simulink model "sm_cvt_power_split_pg_4range"  (R2025a)
settings: Solver=daessc  StartTime=0.0  StopTime=cvtPar.ratioInp.t(end)  MaxStep=0.01  RelTol=1e-3  AbsTol=1e-4  EnableMultiTasking=on
PreLoadFcn:
  | cvtPar = sm_cvt_power_split_pg_4range_param('InputOutput', HMPST);
PostLoadFcn:
  | set_param([bdroot '/Manual Switch'], 'sw', '1')
StartFcn:
  | tic
StopFcn:
  | Elapsed_Sim_Time = toc;
  | disp(['Elapsed Sim Time = ' num2str(Elapsed_Sim_Time)]);
values from neighbouring files (symbols this model uses):
  HMPST = varargin{2}    [sm_cvt_power_split_pg_4range_param.m]
undefined symbols (not defined in the file or in its folder): Local, X, Y, Z
libraries: sm_lib x37, fl_lib x22, nesl_utility x10, planetary_gear_lib x9, Multibody_Parts_Lib x8, simulink x2, sm_wheel_loader_lib x1
(part 1 of 2)
CloseFcn:
  | try,close(h1_sm_planetary_gear_testrig),end
  | clear h1_sm_planetary_gear_testrig
  | 
  | clear simlog_sm_planetary_gear_testrig
  | clear logsout_sm_planetary_gear_testrig
Description:
  | Power Split CVT with Four Speed Ranges
  | 
  | Copyright 2023-2025 The MathWorks, Inc.
settings Model: Creator=smiller  LastModifiedBy=smiller
settings SolverCC: AutoScaleAbsTol=off  AlgebraicLoopSolver=TrustRegion
settings DataIOCC: MaxDataPoints=20000  SaveFormat=Array  ReturnWorkspaceOutputs=off  SignalLoggingName=logsout_sm_cvt_power_split_pg_4range
settings OptimizationCC: ReuseModelBlockBuffer=off  LifeSpan=inf
settings DebuggingCC: UnderspecifiedInitializationDetection=Classic  MergeDetectMultiDrivingBlocksExec=none  SolverPrmCheckMsg=warning  UnconnectedInputMsg=warning  UnconnectedOutputMsg=warning  UnconnectedLineMsg=warning  StateNameClashWarn=warning  PregeneratedLibrarySubsystemCodeDiagnostic=none  SFUnexpectedBacktrackingDiag=warning  SFNoUnconditionalDefaultTransitionDiag=warning  SFExecutionAtInitializationDiag=none  ArithmeticOperatorsInVariantConditions=warning
settings HardwareCC: ProdBitPerPointer=32.0  ProdBitPerSizeT=32.0  ProdBitPerPtrDiffT=32.0  ProdLargestAtomicFloat=None  ProdIntDivRoundTo=Undefined  ProdEndianess=Unspecified  ProdWordSize=32.0  ProdHWDeviceType=32-bit Generic
settings ModelReferenceCC: EnableRefExpFcnMdlSchedulingChecks=on  PropagateSignalLabelsOutOfModel=off
settings SFSimCC: SimUseLocalCustomCode=off  CustomCodeUndefinedFunction=UseInterfaceOnly
settings RTWCC: RTWUseLocalCustomCode=off  GPUComputeCapability=3.5  DLArmComputeVersion=19.05
settings CodeAppCC: StateflowObjectComments=on
settings GRTTargetCC: TargetLangStandard=C89/C90 (ANSI)
settings ConfigComp: CovMetricSettings=dw  CovSaveCumulativeToWorkspaceVar=on  CovSaveSingleToWorkspaceVar=on  CovExternalEMLEnable=off
settings SimscapeCC: SimscapeNormalizeSystem=off  SimscapeLogType=all  SimscapeLogSimulationStatistics=on  SimscapeLogName=simlog_sm_cvt_power_split_pg_4range  SimscapeLogLimitData=off  SimscapeLogDataHistory=20000.0
settings ConfigurationSet: Description=SimMechanics 2G
settings DiagnosticsConfigSet: SimMechanicsUnconnectedFramePorts=none
settings ExplorerConfigSet: InternalSimMechanicsExplorerSettings="<ExplorerConfiguration><canonicalview>default</canonicalview><AnimationSetting><BasePlaybackSpeed>1.0</BasePlaybackSpeed><PlaybackSpeedFactor>2.0</PlaybackSpeedFactor></AnimationSetting><TilePanel><TileInfo><Tiles Columns=\"1\" Count=\"1\" Rows=\"1\"><Column Weight=\"1\"/><Row Weight=\"1\"/><Tile Height=\"1\" Width=\"1\" X=\"0\" Y=\"0\"/></Tiles></TileInfo><SceneInfo><SceneViewer><BGColor><R>1</R><G>1</G><B>1</B></BGColor><Camera><DoPerspective>off</DoPerspective><Position><X>0.0480133750302565443</X><Y>0.998189165564586478</Y><Z>0.410806874332134753</Z></Position><Center><X>0.0475311378746693936</X><Y>0.0361071202127969879</Y><Z>0.138047079899298764</Z></Center><Up><X>0.999999473002182615</X><Y>-0.000216739834242075458</Y><Z>-0.0010035034634835007</Z></Up><ViewLimDist>1</ViewLimDist><YLim>0.276201890267888606</YLim><XLim>0.56263348017532866</XLim></Camera></SceneViewer></SceneInfo></TilePanel><MechEditorPanel><Cameras/><GfxPanelCameraMap/><VideoCreator><PlaybackSpeedRatio>2</PlaybackSpeedRatio><FrameRate>30</FrameRate><VideoFormat>MPEG-4</VideoFormat><FrameSize>auto</FrameSize></VideoCreator></MechEditorPanel></ExplorerConfiguration>"

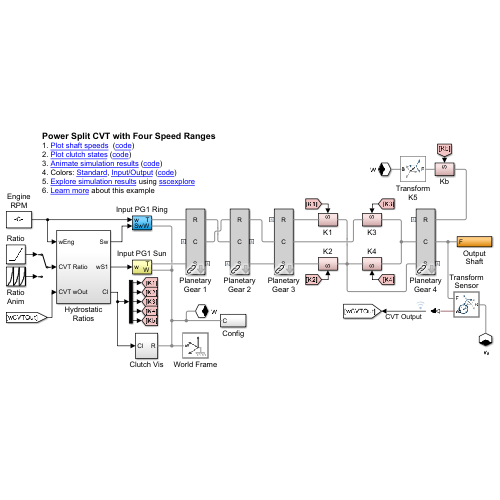
[thumbnail: Simulink's stored preview of the top-level diagram]
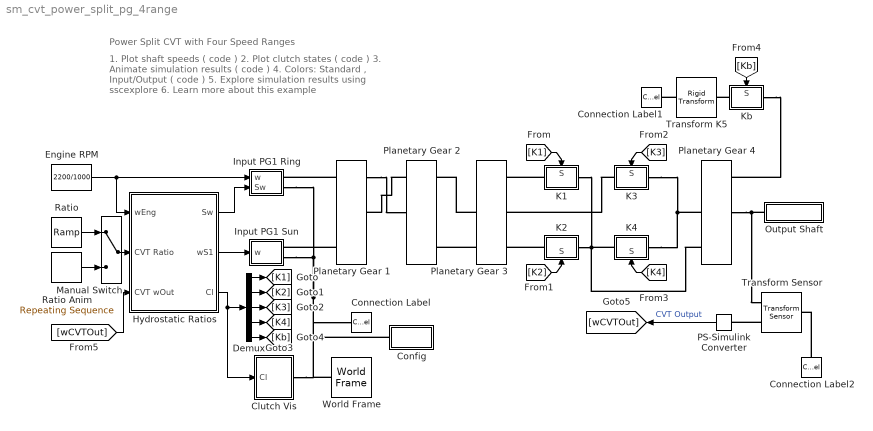
== system sm_cvt_power_split_pg_4range ==
  note: Power Split CVT with Four Speed Ranges
  note: 1. Plot shaft speeds ( code )
      | 2. Plot clutch states ( code )
      | 3. Animate simulation results ( code )
      | 4. Colors: Standard , Input/Output ( code )
      | 5. Explore simulation results using sscexplore
      | 6. Learn more about this example
  Clutch Vis : Subsystem
  Config : Subsystem
  Connection Label : ConnectionLabel  Label=W
  Connection Label1 : ConnectionLabel  Label=W
  Connection Label2 : ConnectionLabel  Label=W
  Demux : Demux  Outputs=5
  Engine RPM : Constant  Value=2200/1000
  Hydrostatic Ratios : Subsystem
  Input PG1 Ring : Subsystem  Tag=PublishSubsystem
  Input PG1 Sun : Subsystem  Tag=PublishSubsystem
  K1 : Subsystem
      settings: PortSchema="{\"entries\":[{\"content\":{\"sides\":[{\"content\":{\"connectorIds\":[\"LConn1\"]},\"type\":\"ConnectorPlacement.EquallySpacedRectSide\",\"uuid\":\"8540058f-cef1-4155-b235-6fcdc2adbf7a\"},{\"content\":{\"connectorIds\":[\"RConn1\"],\"side\":\"RIGHT\"},\"type\":\"ConnectorPlacement.EquallySpacedRectSide\",\"uuid\":\"a5955f9a-e2a5-407c-ab0f-07844d9b5a94\"},{\"content\":{\"connectorIds\":[\"In1\"],\"side\":\"TOP\"},\"type\":\"ConnectorPlacement.EquallySpacedRectSide\",\"uuid\":\"6ad60a3a-82ac-4ebb-acab-e8d6af80f4b1\"}]},\"type\":\"ConnectorPlacement.EquallySpacedConnector\",\"uuid\":\"9d3f1ab8-7892-4728-ac99-ab2f347c5259\"}],\"packageUris\":[\"http://schema.mathworks.com/mf0/Connector/R2020b\"],\"version\":\"1.0\"}"
  K2 : Subsystem
      settings: PortSchema="{\"entries\":[{\"content\":{\"sides\":[{\"content\":{\"connectorIds\":[\"LConn1\"]},\"type\":\"ConnectorPlacement.EquallySpacedRectSide\",\"uuid\":\"8540058f-cef1-4155-b235-6fcdc2adbf7a\"},{\"content\":{\"connectorIds\":[\"RConn1\"],\"side\":\"RIGHT\"},\"type\":\"ConnectorPlacement.EquallySpacedRectSide\",\"uuid\":\"a5955f9a-e2a5-407c-ab0f-07844d9b5a94\"},{\"content\":{\"connectorIds\":[\"In1\"],\"side\":\"TOP\"},\"type\":\"ConnectorPlacement.EquallySpacedRectSide\",\"uuid\":\"6ad60a3a-82ac-4ebb-acab-e8d6af80f4b1\"}]},\"type\":\"ConnectorPlacement.EquallySpacedConnector\",\"uuid\":\"9d3f1ab8-7892-4728-ac99-ab2f347c5259\"}],\"packageUris\":[\"http://schema.mathworks.com/mf0/Connector/R2020b\"],\"version\":\"1.0\"}"
  K3 : Subsystem
      settings: PortSchema="{\"entries\":[{\"content\":{\"sides\":[{\"content\":{\"connectorIds\":[\"LConn1\"]},\"type\":\"ConnectorPlacement.EquallySpacedRectSide\",\"uuid\":\"8540058f-cef1-4155-b235-6fcdc2adbf7a\"},{\"content\":{\"connectorIds\":[\"RConn1\"],\"side\":\"RIGHT\"},\"type\":\"ConnectorPlacement.EquallySpacedRectSide\",\"uuid\":\"a5955f9a-e2a5-407c-ab0f-07844d9b5a94\"},{\"content\":{\"connectorIds\":[\"In1\"],\"side\":\"TOP\"},\"type\":\"ConnectorPlacement.EquallySpacedRectSide\",\"uuid\":\"6ad60a3a-82ac-4ebb-acab-e8d6af80f4b1\"}]},\"type\":\"ConnectorPlacement.EquallySpacedConnector\",\"uuid\":\"9d3f1ab8-7892-4728-ac99-ab2f347c5259\"}],\"packageUris\":[\"http://schema.mathworks.com/mf0/Connector/R2020b\"],\"version\":\"1.0\"}"
  K4 : Subsystem
      settings: PortSchema="{\"entries\":[{\"content\":{\"sides\":[{\"content\":{\"connectorIds\":[\"LConn1\"]},\"type\":\"ConnectorPlacement.EquallySpacedRectSide\",\"uuid\":\"8540058f-cef1-4155-b235-6fcdc2adbf7a\"},{\"content\":{\"connectorIds\":[\"RConn1\"],\"side\":\"RIGHT\"},\"type\":\"ConnectorPlacement.EquallySpacedRectSide\",\"uuid\":\"a5955f9a-e2a5-407c-ab0f-07844d9b5a94\"},{\"content\":{\"connectorIds\":[\"In1\"],\"side\":\"TOP\"},\"type\":\"ConnectorPlacement.EquallySpacedRectSide\",\"uuid\":\"6ad60a3a-82ac-4ebb-acab-e8d6af80f4b1\"}]},\"type\":\"ConnectorPlacement.EquallySpacedConnector\",\"uuid\":\"9d3f1ab8-7892-4728-ac99-ab2f347c5259\"}],\"packageUris\":[\"http://schema.mathworks.com/mf0/Connector/R2020b\"],\"version\":\"1.0\"}"
  Kb : Subsystem
      settings: PortSchema="{\"entries\":[{\"content\":{\"sides\":[{\"content\":{\"connectorIds\":[\"LConn1\"]},\"type\":\"ConnectorPlacement.EquallySpacedRectSide\",\"uuid\":\"8540058f-cef1-4155-b235-6fcdc2adbf7a\"},{\"content\":{\"connectorIds\":[\"RConn1\"],\"side\":\"RIGHT\"},\"type\":\"ConnectorPlacement.EquallySpacedRectSide\",\"uuid\":\"a5955f9a-e2a5-407c-ab0f-07844d9b5a94\"},{\"content\":{\"connectorIds\":[\"In1\"],\"side\":\"TOP\"},\"type\":\"ConnectorPlacement.EquallySpacedRectSide\",\"uuid\":\"6ad60a3a-82ac-4ebb-acab-e8d6af80f4b1\"}]},\"type\":\"ConnectorPlacement.EquallySpacedConnector\",\"uuid\":\"9d3f1ab8-7892-4728-ac99-ab2f347c5259\"}],\"packageUris\":[\"http://schema.mathworks.com/mf0/Connector/R2020b\"],\"version\":\"1.0\"}"
  Manual Switch : ManualSwitch
  Output Shaft : Subsystem
  PS-Simulink Converter : nesl_utility/PS-Simulink Converter  PhysicalDomain=network_engine_domain  SubClassName=ps_output  LeftPortType=input  RightPortType=output  PseudoPeriodic=off  Frequencies=[]  VectorFormat=inherit  Unit=rpm  AffineConversion=off
  Planetary Gear 1 : planetary_gear_lib/Planetary Gear  Tag=PublishSubsystem  rad_sun=cvtPar.pg1_sun_rad  nteeth_sun=cvtPar.pg1_sun_nteeth  rad_planet=cvtPar.pg1_pla_rad  nteeth_planet=cvtPar.pg1_pla_nteeth  rad_ring=2*cvtPar.pg1_pla_rad+cvtPar.pg1_sun_rad  nteeth_ring=cvtPar.pg1_rin_nteeth  pg_axial_offset=cvtPar.plaGear_axial_offset*1.25  gear_thickness=cvtPar.gear_thickness  link_thickness=cvtPar.link_thickness  rad_hole=cvtPar.rad_hole  ring_gear_clr=cvtPar.clr.pg1.ring  sun_gear_clr=cvtPar.clr.pg1.sun  pla_gear_clr=cvtPar.clr.pg1.pla  carrier_color=cvtPar.clr.pg1.carr
  Planetary Gear 2 : planetary_gear_lib/Planetary Gear  Tag=PublishSubsystem  rad_sun=cvtPar.pg2_sun_rad  nteeth_sun=cvtPar.pg2_sun_nteeth  rad_planet=cvtPar.pg2_pla_rad  nteeth_planet=cvtPar.pg2_pla_nteeth  rad_ring=2*cvtPar.pg2_pla_rad+cvtPar.pg2_sun_rad  nteeth_ring=cvtPar.pg2_rin_nteeth  pg_axial_offset=cvtPar.plaGear_axial_offset*1.25  gear_thickness=cvtPar.gear_thickness  link_thickness=cvtPar.link_thickness  rad_hole=cvtPar.rad_hole  ring_gear_clr=cvtPar.clr.pg2.ring  sun_gear_clr=cvtPar.clr.pg2.sun  pla_gear_clr=cvtPar.clr.pg2.pla  carrier_color=cvtPar.clr.pg2.carr
  Planetary Gear 3 : planetary_gear_lib/Planetary Gear  Tag=PublishSubsystem  rad_sun=cvtPar.pg3_sun_rad  nteeth_sun=cvtPar.pg3_sun_nteeth  rad_planet=cvtPar.pg3_pla_rad  nteeth_planet=cvtPar.pg3_pla_nteeth  rad_ring=2*cvtPar.pg3_pla_rad+cvtPar.pg3_sun_rad  nteeth_ring=cvtPar.pg3_rin_nteeth  pg_axial_offset=cvtPar.plaGear_axial_offset*3  gear_thickness=cvtPar.gear_thickness  link_thickness=cvtPar.link_thickness  rad_hole=cvtPar.rad_hole  ring_gear_clr=cvtPar.clr.pg3.ring  sun_gear_clr=cvtPar.clr.pg3.sun  pla_gear_clr=cvtPar.clr.pg3.pla  carrier_color=cvtPar.clr.pg3.carr
  Planetary Gear 4 : planetary_gear_lib/Planetary Gear  Tag=PublishSubsystem  rad_sun=cvtPar.pg4_sun_rad  nteeth_sun=cvtPar.pg4_sun_nteeth  rad_planet=cvtPar.pg4_pla_rad  nteeth_planet=cvtPar.pg4_pla_nteeth  rad_ring=2*cvtPar.pg4_pla_rad+cvtPar.pg4_sun_rad  nteeth_ring=cvtPar.pg4_rin_nteeth  pg_axial_offset=cvtPar.plaGear_axial_offset  gear_thickness=cvtPar.gear_thickness  link_thickness=cvtPar.link_thickness  rad_hole=cvtPar.rad_hole  ring_gear_clr=cvtPar.clr.pg4.ring  sun_gear_clr=cvtPar.clr.pg4.sun  pla_gear_clr=cvtPar.clr.pg4.pla  carrier_color=cvtPar.clr.pg4.carr
  Ratio : simulink/Sources/Ramp  slope=cvtPar.ratioInp.r(end)/(cvtPar.ratioInp.t(end)-20)  start=10  InitialOutput=0
  Ratio Anim : simulink/Sources/Repeating Sequence  rep_seq_t=cvtPar.ratioInp.t  rep_seq_y=cvtPar.ratioInp.r
  Transform K5 : sm_lib/Frames and Transforms/Rigid Transform  RotationMethod=None  FollAlignAxisA=+X  BaseAlignAxisA=+Y  FollAlignAxisB=+Y  BaseAlignAxisB=+Z  RotationStandardAxis=+Z  RotationAngle=0.0  RotationAngleUnits=deg  RotationArbitraryAxis=[0 0 1]  RotationSequenceAxes=FollowerAxes  RotationSequence=XYX  RotationSequenceAngles=[0 0 0]  RotationSequenceAnglesUnits=deg  RotationMatrix=[1 0 0; 0 1 0; 0 0 1]  Quaternion=[1 0 0 0]  TranslationMethod=StandardAxis  TranslationCartesianOffset=[0 0 0]  TranslationCartesianOffsetUnits=m  TranslationStandardAxis=+Z  TranslationStandardOffset=cvtPar.plaGear_axial_offset*6.5  TranslationStandardOffsetUnits=m  TranslationROffset=0  TranslationROffsetUnits=m  TranslationThetaOffset=0  TranslationThetaOffsetUnits=deg  TranslationZOffset=0  TranslationZOffsetUnits=m
  Transform Sensor : sm_lib/Frames and Transforms/Transform Sensor  MeasurementFrame=World  RotationSequence=XYX  SenseAngle=off  SenseAxis=off  SenseQ=off  SenseR=off  SenseRotationSequence=off  SenseOmegaX=off  SenseOmegaY=off  SenseOmegaZ=on  SenseOmega=off  SenseQDot=off  SenseRDot=off  SenseRotationSequenceDot=off  SenseAlphaX=off  SenseAlphaY=off  SenseAlphaZ=off  SenseAlpha=off  SenseQDDot=off  SenseRDDot=off  SenseX=off  SenseY=off  SenseZ=off  SenseXYZ=off  SenseRad=off  SenseAzim=off  SenseDist=off  SenseInc=off  SenseXDot=off  SenseYDot=off  SenseZDot=off  SenseXYZDot=off  SenseRadDot=off  SenseAzimDot=off  SenseDistDot=off  SenseIncDot=off  SenseXDDot=off  SenseYDDot=off  SenseZDDot=off  SenseXYZDDot=off  SenseRadDDot=off  SenseAzimDDot=off  SenseDistDDot=off  SenseIncDDot=off
  World Frame : sm_lib/Frames and Transforms/World Frame
  wires:
  Engine RPM/1 -> Input PG1 Ring/1(w), Hydrostatic Ratios/1(wEng)
  [K1] -> K1/1(S)
  [K2] -> K2/1(S)
  [K3] -> K3/1(S)
  [K4] -> K4/1(S)
  [Kb] -> Kb/1(S)
  Demux/3 -> [K3]
  Demux/4 -> [K4]
  Demux/5 -> [Kb]
  Demux/1 -> [K1]
  Demux/2 -> [K2]
  Manual Switch/1 -> Hydrostatic Ratios/2(CVT Ratio)
  PS-Simulink Converter/1 -> [wCVTOut]  "CVT Output"
  Hydrostatic Ratios/2(wS1) -> Input PG1 Sun/1(w)
  Hydrostatic Ratios/3(Cl) -> Clutch Vis/1(Cl), Demux/1
  [wCVTOut] -> Hydrostatic Ratios/3(CVT wOut)
  Hydrostatic Ratios/1(Sw) -> Input PG1 Ring/2(Sw)
  Ratio Anim/1 -> Manual Switch/2
  Ratio/1 -> Manual Switch/1
  connections:
  Planetary Gear 1/LConn3 -- Input PG1 Sun/RConn1
  Planetary Gear 1/LConn1 -- Input PG1 Ring/RConn1
  Planetary Gear 1/RConn1 -- Planetary Gear 2/LConn2
  Planetary Gear 2/LConn1 -- Planetary Gear 1/RConn2
  Planetary Gear 3/LConn2 -- Planetary Gear 2/RConn1
  Planetary Gear 3/LConn3 -- Planetary Gear 2/RConn3
  K1/LConn1 -- Planetary Gear 3/RConn1
  Planetary Gear 4/LConn3 -- K4/LConn1 -- K2/RConn1 -- K1/RConn1
  K2/LConn1 -- Planetary Gear 3/RConn3
  Planetary Gear 4/LConn2 -- K4/RConn1 -- K3/LConn1
  Kb/LConn1 -- Planetary Gear 4/RConn1
  Kb/RConn1 -- Transform K5/RConn1
  Transform K5/LConn1 -- Connection Label1/LConn1
  K3/RConn1 -- Planetary Gear 3/RConn2
  Planetary Gear 4/RConn2 -- Output Shaft/RConn1 -- Transform Sensor/RConn1
  Connection Label2/LConn1 -- Transform Sensor/LConn1
  Transform Sensor/RConn2 -- PS-Simulink Converter/LConn1
  Input PG1 Ring/RConn2 -- Config/LConn1 -- Connection Label/LConn1 -- World Frame/RConn1 -- Clutch Vis/RConn1 -- Input PG1 Sun/RConn2

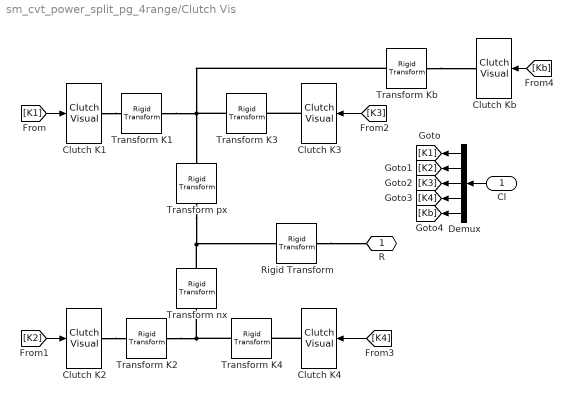
== system sm_cvt_power_split_pg_4range/Clutch Vis ==
  Cl : Inport
  Clutch K{1..4} (4 alike) : planetary_gear_lib/Clutch Visual  SystemSampleTime=-1  VariantActivationTime=update diagram  EmptyChoice=off  PassThrough=off  PassThroughVariantControl=(default)  EmptyChoiceVariantControl=(default)  AllowFlexibleInterface=on  Latency=0  AutoFrameSizeCalculation=off
  Clutch Kb : planetary_gear_lib/Clutch Visual  SystemSampleTime=-1  VariantActivationTime=update diagram  EmptyChoice=off  PassThrough=off  PassThroughVariantControl=(default)  EmptyChoiceVariantControl=(default)  AllowFlexibleInterface=on  Latency=0  AutoFrameSizeCalculation=off
  Demux : Demux  Outputs=5
  Rigid Transform : sm_lib/Frames and Transforms/Rigid Transform  RotationMethod=None  FollAlignAxisA=+X  BaseAlignAxisA=+Y  FollAlignAxisB=+Y  BaseAlignAxisB=+Z  RotationStandardAxis=+Z  RotationAngle=0.0  RotationAngleUnits=deg  RotationArbitraryAxis=[0 0 1]  RotationSequenceAxes=FollowerAxes  RotationSequence=XYX  RotationSequenceAngles=[0 0 0]  RotationSequenceAnglesUnits=deg  RotationMatrix=[1 0 0; 0 1 0; 0 0 1]  Quaternion=[1 0 0 0]  TranslationMethod=StandardAxis  TranslationCartesianOffset=[0 0 0]  TranslationCartesianOffsetUnits=m  TranslationStandardAxis=+Z  TranslationStandardOffset=cvtPar.plaGear_axial_offset*4  TranslationStandardOffsetUnits=m  TranslationROffset=0  TranslationROffsetUnits=m  TranslationThetaOffset=0  TranslationThetaOffsetUnits=deg  TranslationZOffset=0  TranslationZOffsetUnits=m
  Transform K{1..4} (4 alike) : sm_lib/Frames and Transforms/Rigid Transform  RotationMethod=None  FollAlignAxisA=+X  BaseAlignAxisA=+Y  FollAlignAxisB=+Y  BaseAlignAxisB=+Z  RotationStandardAxis=+Z  RotationAngle=0.0  RotationAngleUnits=deg  RotationArbitraryAxis=[0 0 1]  RotationSequenceAxes=FollowerAxes  RotationSequence=XYX  RotationSequenceAngles=[0 0 0]  RotationSequenceAnglesUnits=deg  RotationMatrix=[1 0 0; 0 1 0; 0 0 1]  Quaternion=[1 0 0 0]  TranslationMethod=StandardAxis  TranslationCartesianOffset=[0 0 0]  TranslationCartesianOffsetUnits=m  TranslationStandardAxis=+Z  TranslationStandardOffset=cvtPar.plaGear_axial_offset/3  TranslationStandardOffsetUnits=m  TranslationROffset=0  TranslationROffsetUnits=m  TranslationThetaOffset=0  TranslationThetaOffsetUnits=deg  TranslationZOffset=0  TranslationZOffsetUnits=m
  Transform Kb : sm_lib/Frames and Transforms/Rigid Transform  RotationMethod=None  FollAlignAxisA=+X  BaseAlignAxisA=+Y  FollAlignAxisB=+Y  BaseAlignAxisB=+Z  RotationStandardAxis=+Z  RotationAngle=0.0  RotationAngleUnits=deg  RotationArbitraryAxis=[0 0 1]  RotationSequenceAxes=FollowerAxes  RotationSequence=XYX  RotationSequenceAngles=[0 0 0]  RotationSequenceAnglesUnits=deg  RotationMatrix=[1 0 0; 0 1 0; 0 0 1]  Quaternion=[1 0 0 0]  TranslationMethod=StandardAxis  TranslationCartesianOffset=[0 0 0]  TranslationCartesianOffsetUnits=m  TranslationStandardAxis=+Z  TranslationStandardOffset=cvtPar.plaGear_axial_offset*2.5  TranslationStandardOffsetUnits=m  TranslationROffset=0  TranslationROffsetUnits=m  TranslationThetaOffset=0  TranslationThetaOffsetUnits=deg  TranslationZOffset=0  TranslationZOffsetUnits=m
  Transform nx : sm_lib/Frames and Transforms/Rigid Transform  RotationMethod=None  FollAlignAxisA=+X  BaseAlignAxisA=+Y  FollAlignAxisB=+Y  BaseAlignAxisB=+Z  RotationStandardAxis=+Z  RotationAngle=0.0  RotationAngleUnits=deg  RotationArbitraryAxis=[0 0 1]  RotationSequenceAxes=FollowerAxes  RotationSequence=XYX  RotationSequenceAngles=[0 0 0]  RotationSequenceAnglesUnits=deg  RotationMatrix=[1 0 0; 0 1 0; 0 0 1]  Quaternion=[1 0 0 0]  TranslationMethod=StandardAxis  TranslationCartesianOffset=[0 0 0]  TranslationCartesianOffsetUnits=m  TranslationStandardAxis=+X  TranslationStandardOffset=(2*cvtPar.pg3_pla_rad+cvtPar.pg3_sun_rad)*0.75  TranslationStandardOffsetUnits=m  TranslationROffset=0  TranslationROffsetUnits=m  TranslationThetaOffset=0  TranslationThetaOffsetUnits=deg  TranslationZOffset=0  TranslationZOffsetUnits=m
  Transform px : sm_lib/Frames and Transforms/Rigid Transform  RotationMethod=None  FollAlignAxisA=+X  BaseAlignAxisA=+Y  FollAlignAxisB=+Y  BaseAlignAxisB=+Z  RotationStandardAxis=+Z  RotationAngle=0.0  RotationAngleUnits=deg  RotationArbitraryAxis=[0 0 1]  RotationSequenceAxes=FollowerAxes  RotationSequence=XYX  RotationSequenceAngles=[0 0 0]  RotationSequenceAnglesUnits=deg  RotationMatrix=[1 0 0; 0 1 0; 0 0 1]  Quaternion=[1 0 0 0]  TranslationMethod=StandardAxis  TranslationCartesianOffset=[0 0 0]  TranslationCartesianOffsetUnits=m  TranslationStandardAxis=+X  TranslationStandardOffset=(2*cvtPar.pg3_pla_rad+cvtPar.pg3_sun_rad)*0.75  TranslationStandardOffsetUnits=m  TranslationROffset=0  TranslationROffsetUnits=m  TranslationThetaOffset=0  TranslationThetaOffsetUnits=deg  TranslationZOffset=0  TranslationZOffsetUnits=m
  R : PMIOPort  Side=Right
  wires:
  Cl/1 -> Demux/1
  Demux/1 -> [K1]
  Demux/3 -> [K3]
  Demux/2 -> [K2]
  Demux/4 -> [K4]
  Demux/5 -> [Kb]
  [K1] -> Clutch K1/1
  [K2] -> Clutch K2/1
  [K3] -> Clutch K3/1
  [K4] -> Clutch K4/1
  [Kb] -> Clutch Kb/1
  connections:
  Rigid Transform/LConn1 -- R/RConn1
  Transform K3/LConn1 -- Transform Kb/LConn1 -- Transform K1/RConn1 -- Transform px/RConn1
  Transform px/LConn1 -- Transform nx/RConn1 -- Rigid Transform/RConn1
  Transform K4/LConn1 -- Transform K2/RConn1 -- Transform nx/LConn1
  Clutch K3/RConn1 -- Transform K3/RConn1
  Clutch K1/RConn1 -- Transform K1/LConn1
  Clutch K2/RConn1 -- Transform K2/LConn1
  Clutch K4/RConn1 -- Transform K4/RConn1
  Transform Kb/RConn1 -- Clutch Kb/RConn1

== system sm_cvt_power_split_pg_4range/Config ==
  Mechanism Configuration : sm_lib/Utilities/Mechanism Configuration  UniformGravity=Constant  GravityVector=[0 0 0]  GravityVectorUnits=m/s^2  LinearizationDelta=0.001  JointModeTransitionNonlinearIterations=2
  Solver Configuration : nesl_utility/Solver Configuration  PhysicalDomain=network_engine_domain  SubClassName=solver  LeftPortType=input  RightPortType=generic  Tones=[]  Harmonics=[]  SimulateNoise=off  Profile=off  UseLocalSampling=off  EnableSwitchedLinearOptims=on  FrequencyDomain=off  UseCCode=off  RelTol=0.001  AbsTol=1e-06  MinStep=1e-09  ToWorkspace=off  RevertToSquareIcSolve=off  NumHomotopyIterations=100  PhasorMode=off  PhasorModeNumHarmonics=1  ConsistencySolver=NEWTON_FTOL  IndexReductionMethod=DerivativeReplacement  DoDC=off  ResidualTolerance=1e-9  ConsistencyTolSource=GLOBAL  ConsistencyAbsTol=0.001  ConsistencyRelTol=0.001  ConsistencyTolFactor=0.001  UseLocalSolver=off  LocalSolverChoice=NE_BACKWARD_EULER_ADVANCER  ResolveIndetEquations=on  FunctionEvalNumThread=1  LocalSolverSampleTime=.001  DoFixedCost=off  MaxNonlinIter=3  MaxModeIter=2  ComputeImpulses=off  ImpulseIterations=2  LinearAlgebra=Sparse  LinearAlgebraNumThread=0  EquationFormulation=NE_TIME_EF  DelaysMemoryBudget=1024  AutomaticFiltering=on  FilteringTimeConstant=0.001  PartitionStorageMethod=AS_NEEDED  PartitionMemoryBudget=1024  PartitionMethod=FAST  MultibodyUseLocalSolver=off  MultibodyLocalSolverChoice=ODE1  MultibodyLocalSolverSampleTime=0.001
  C : PMIOPort  Side=Left
  connections:
  Mechanism Configuration/RConn1 -- Solver Configuration/RConn1 -- C/RConn1

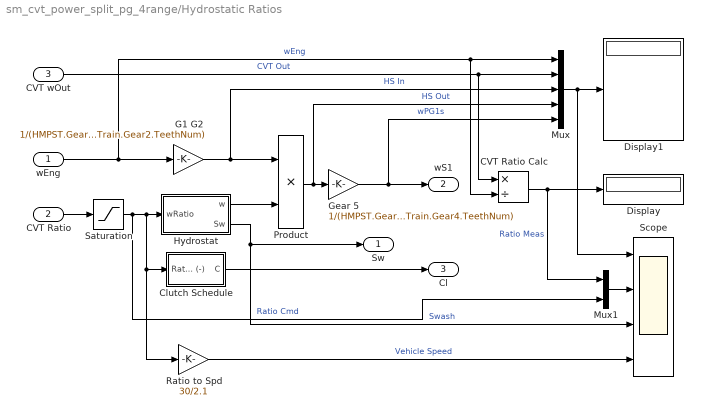
== system sm_cvt_power_split_pg_4range/Hydrostatic Ratios ==
  wEng : Inport
  CVT Ratio : Inport  Port=2
  CVT wOut : Inport  Port=3
  CVT Ratio Calc : Product  Inputs=*/
  Clutch Schedule : Subsystem
  Display : Display
  Display1 : Display
  G1 G2 : Gain  Gain=1/(HMPST.GearTrain.Gear2.TeethNum/HMPST.GearTrain.Gear1.TeethNum*HMPST.GearTrain.Gear3.TeethNum/HMPST.GearTrain.Gear2.TeethNum)
  Gear 5 : Gain  Gain=1/(HMPST.GearTrain.Gear5.TeethNum/HMPST.GearTrain.Gear4.TeethNum)
  Hydrostat : Subsystem
  Mux : Mux  Inputs=5
  Mux1 : Mux  Inputs=2
  Product : Product
  Ratio to Spd : Gain  Gain=30/2.1
  Saturation : Saturate  UpperLimit=2.1  ZeroCross=off
  Scope : Scope  NumInputPorts=4
      settings: ActiveDisplayYMinimum=-4.0523  ActiveDisplayYMaximum=5.54315
  Sw : Outport
  wS1 : Outport  Port=2
  Cl : Outport  Port=3
  wires:
  Clutch Schedule/1(C) -> Cl/1
  Ratio to Spd/1 -> Scope/4  "Vehicle Speed"
  Saturation/1 -> Mux1/2, Ratio to Spd/1, Clutch Schedule/1(Ratio (-)), Hydrostat/1(wRatio)  "Ratio Cmd"
  Hydrostat/2(Sw) -> Scope/3, Sw/1  "Swash"
  wEng/1 -> Mux/1, CVT Ratio Calc/2, G1 G2/1  "wEng"
  CVT Ratio Calc/1 -> Display/1, Mux1/1  "Ratio Meas"
  Mux/1 -> Display1/1, Scope/1
  CVT wOut/1 -> Mux/2, CVT Ratio Calc/1  "CVT Out"
  Gear 5/1 -> Mux/5, wS1/1  "wPG1s"
  CVT Ratio/1 -> Saturation/1
  Product/1 -> Mux/4, Gear 5/1  "HS Out"
  G1 G2/1 -> Mux/3, Product/1  "HS In"
  Hydrostat/1(w) -> Product/2
  Mux1/1 -> Scope/2

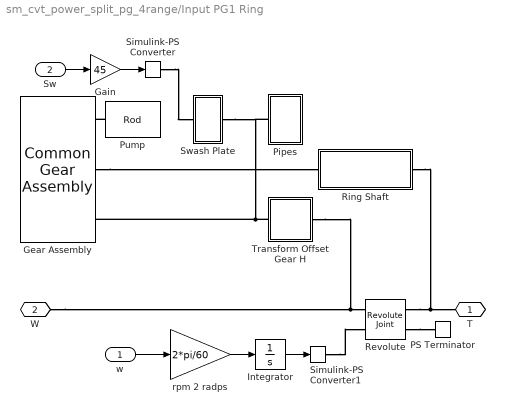
== system sm_cvt_power_split_pg_4range/Input PG1 Ring ==
  w : Inport
  Sw : Inport  Port=2
  Gain : Gain  Gain=45
  Gear Assembly : Multibody_Parts_Lib/Gears/Assemblies/Common Gear Assembly  Tag=PublishSubsystem  b_gear_pd_asy=0.225  f_gear_pd_asy=0.15  b_gear_nt=36  f_gear_nt=24  b_gear_th=0.02  f_gear_th=0.02  f_popup_gear_type=External  b_gear_rh=0.01  f_gear_rht=0.01  b_gear_offset_angle=0  f_gear_offset_angle=360/24/2  b_gear_rho=7000  f_gear_rho=7000  b_gear_clr=cvtPar.clr.pg1.ring  f_gear_clr=[1.0 0.6 0.0]*0+[0.2 0.6 0.2]  b_gear_opc=1  f_gear_opc=1  popup_ad_dd_asy=Specify  b_gear_ad=0.225/36  f_gear_ad=0.15/24  b_gear_dd=1.157*0.225/36  f_gear_dd=1.157*0.15/24  b_visc_frict_asy=0.01  f_visc_frict_asy=0.01  b_popup_markings=Two  f_popup_markings=Two  b_mark_radius_range=[0.6 0.7]  f_mark_radius_range=[0.7 0.8]  b_mark_angle_range=60  f_mark_angle_range=60  b_mark_color=[1 1 1]  f_mark_color=[1 1 1]
  Integrator : Integrator
  PS Terminator : fl_lib/Physical Signals/Sinks/PS Terminator
  Pipes : Subsystem
  Pump : Multibody_Parts_Lib/Basic/Rod  rod_rad=0.025*2  rod_len=0.05*2  rod_rho=7000  rod_color=[1.0 0.6 0.0]*0+[0.2 0.6 0.2]  rod_opc=0.5  popup_zori=Local +Z  popup_markings=Two  mark_radius_range=[0.5 0.75]  mark_length_range=1.005  mark_angle_range=15  mark_color=[1 1 1]
  Revolute : sm_lib/Joints/Revolute Joint  JointMode=Normal  CompositeWrenchDir=FollowerOnBase  CompositeWrenchFrame=BaseFrame  SenseConstraintForce=off  SenseConstraintTorque=off  SenseTotalForce=off  SenseTotalTorque=off  PositionTargetSpecify=off  PositionTargetPriority=High  PositionTargetValue=0  PositionTargetValueUnits=deg  VelocityTargetSpecify=off  VelocityTargetPriority=High  VelocityTargetValue=0  VelocityTargetValueUnits=deg/s  EquilibriumPosition=0  EquilibriumPositionUnits=deg  SpringStiffness=0  SpringStiffnessUnits=N*m/deg  DampingCoefficient=0  DampingCoefficientUnits=N*m/(deg/s)  LowerLimitSpecify=off  LowerLimitBound=-90  LowerLimitBoundUnits=deg  LowerLimitStiffness=1e4  LowerLimitStiffnessUnits=N*m/deg  LowerLimitDamping=10  LowerLimitDampingUnits=N*m/(deg/s)  LowerLimitTransitionRegionWidth=0.1  LowerLimitTransitionRegionWidthUnits=deg  UpperLimitSpecify=off  UpperLimitBound=90  UpperLimitBoundUnits=deg  UpperLimitStiffness=1e4  UpperLimitStiffnessUnits=N*m/deg  UpperLimitDamping=10  UpperLimitDampingUnits=N*m/(deg/s)  UpperLimitTransitionRegionWidth=0.1  UpperLimitTransitionRegionWidthUnits=deg  TorqueActuationMode=ComputedTorque  MotionActuationMode=InputMotion  SensePosition=off  SenseVelocity=on  SenseAcceleration=off  SenseTorqueForce=off  SenseLowerLimitTorqueForce=off  SenseUpperLimitTorqueForce=off
  Ring Shaft : Subsystem
  Simulink-PS Converter : nesl_utility/Simulink-PS Converter  PhysicalDomain=network_engine_domain  SubClassName=ps_input  LeftPortType=input  RightPortType=output  PseudoPeriodic=off  Frequencies=[]  NoiseDistribution=none  NoiseParameters=[]  Unit=deg  AffineConversion=off  FilteringAndDerivatives=filter  SimscapeFilterOrder=2  InputFilterTimeConstant=0.001  UdotUserProvided=0
  Simulink-PS Converter1 : nesl_utility/Simulink-PS Converter  PhysicalDomain=network_engine_domain  SubClassName=ps_input  LeftPortType=input  RightPortType=output  PseudoPeriodic=off  Frequencies=[]  NoiseDistribution=none  NoiseParameters=[]  Unit=rad  AffineConversion=off  FilteringAndDerivatives=filter  SimscapeFilterOrder=2  InputFilterTimeConstant=0.001  UdotUserProvided=0
  Swash Plate : Subsystem
  Transform Offset Gear H : Subsystem
  rpm 2 radps : Gain  Gain=2*pi/60
  T : PMIOPort  Side=Right
  W : PMIOPort  Port=2  Side=Right
  wires:
  Integrator/1 -> Simulink-PS Converter1/1
  w/1 -> rpm 2 radps/1
  rpm 2 radps/1 -> Integrator/1
  Sw/1 -> Gain/1
  Gain/1 -> Simulink-PS Converter/1
  connections:
  Simulink-PS Converter1/RConn1 -- Revolute/LConn2
  Revolute/RConn2 -- PS Terminator/LConn1
  Revolute/RConn1 -- Ring Shaft/RConn1 -- T/RConn1
  Pump/LConn1 -- Gear Assembly/LConn1
  W/RConn1 -- Transform Offset Gear H/RConn1 -- Revolute/LConn1
  Transform Offset Gear H/LConn1 -- Pipes/RConn1 -- Swash Plate/RConn1 -- Gear Assembly/LConn3
  Simulink-PS Converter/RConn1 -- Swash Plate/LConn1
  Gear Assembly/LConn2 -- Ring Shaft/LConn1

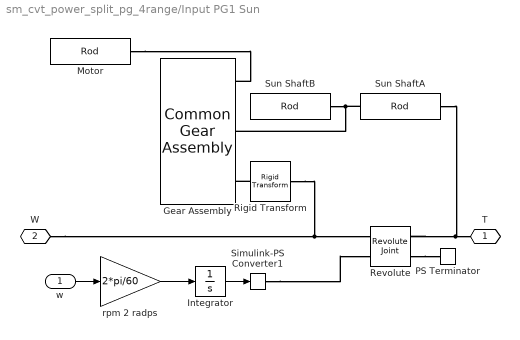
== system sm_cvt_power_split_pg_4range/Input PG1 Sun ==
  w : Inport
  Gear Assembly : Multibody_Parts_Lib/Gears/Assemblies/Common Gear Assembly  Tag=PublishSubsystem  b_gear_pd_asy=0.125  f_gear_pd_asy=0.25  b_gear_nt=20  f_gear_nt=40  b_gear_th=0.02  f_gear_th=0.02  f_popup_gear_type=External  b_gear_rh=0.01  f_gear_rht=0.01  b_gear_offset_angle=0  f_gear_offset_angle=360/24/2  b_gear_rho=7000  f_gear_rho=7000  b_gear_clr=cvtPar.clr.pg1.sun  f_gear_clr=cvtPar.clr.pg1.sun*0+[0.4 0.4 1.0]  b_gear_opc=1  f_gear_opc=1  popup_ad_dd_asy=Specify  b_gear_ad=0.125/20  f_gear_ad=0.25/40  b_gear_dd=1.157*0.125/20  f_gear_dd=1.157*0.25/40  b_visc_frict_asy=0.01  f_visc_frict_asy=0.01  b_popup_markings=Two  f_popup_markings=Two  b_mark_radius_range=[0.6 0.7]  f_mark_radius_range=[0.7 0.8]  b_mark_angle_range=60  f_mark_angle_range=60  b_mark_color=[1 1 1]  f_mark_color=[1 1 1]
  Integrator : Integrator
  Motor : Multibody_Parts_Lib/Basic/Rod  rod_rad=cvtPar.rad_hole*2*5  rod_len=0.1*1  rod_rho=7000  rod_color=[0.2 0.6 0.2]*0+cvtPar.clr.pg1.sun*0+[0.4 0.4 1.0]  rod_opc=0.5  popup_zori=Local +Z  popup_markings=Two  mark_radius_range=[0.5 1.01]  mark_length_range=1.005  mark_angle_range=30  mark_color=[1 1 1]
  PS Terminator : fl_lib/Physical Signals/Sinks/PS Terminator
  Revolute : sm_lib/Joints/Revolute Joint  JointMode=Normal  CompositeWrenchDir=FollowerOnBase  CompositeWrenchFrame=BaseFrame  SenseConstraintForce=off  SenseConstraintTorque=off  SenseTotalForce=off  SenseTotalTorque=off  PositionTargetSpecify=off  PositionTargetPriority=High  PositionTargetValue=0  PositionTargetValueUnits=deg  VelocityTargetSpecify=off  VelocityTargetPriority=High  VelocityTargetValue=0  VelocityTargetValueUnits=deg/s  EquilibriumPosition=0  EquilibriumPositionUnits=deg  SpringStiffness=0  SpringStiffnessUnits=N*m/deg  DampingCoefficient=0  DampingCoefficientUnits=N*m/(deg/s)  LowerLimitSpecify=off  LowerLimitBound=-90  LowerLimitBoundUnits=deg  LowerLimitStiffness=1e4  LowerLimitStiffnessUnits=N*m/deg  LowerLimitDamping=10  LowerLimitDampingUnits=N*m/(deg/s)  LowerLimitTransitionRegionWidth=0.1  LowerLimitTransitionRegionWidthUnits=deg  UpperLimitSpecify=off  UpperLimitBound=90  UpperLimitBoundUnits=deg  UpperLimitStiffness=1e4  UpperLimitStiffnessUnits=N*m/deg  UpperLimitDamping=10  UpperLimitDampingUnits=N*m/(deg/s)  UpperLimitTransitionRegionWidth=0.1  UpperLimitTransitionRegionWidthUnits=deg  TorqueActuationMode=ComputedTorque  MotionActuationMode=InputMotion  SensePosition=off  SenseVelocity=on  SenseAcceleration=off  SenseTorqueForce=off  SenseLowerLimitTorqueForce=off  SenseUpperLimitTorqueForce=off
  Rigid Transform : sm_lib/Frames and Transforms/Rigid Transform  RotationMethod=None  FollAlignAxisA=+X  BaseAlignAxisA=+Y  FollAlignAxisB=+Y  BaseAlignAxisB=+Z  RotationStandardAxis=+Z  RotationAngle=0.0  RotationAngleUnits=deg  RotationArbitraryAxis=[0 0 1]  RotationSequenceAxes=FollowerAxes  RotationSequence=XYX  RotationSequenceAngles=[0 0 0]  RotationSequenceAnglesUnits=deg  RotationMatrix=[1 0 0; 0 1 0; 0 0 1]  Quaternion=[1 0 0 0]  TranslationMethod=StandardAxis  TranslationCartesianOffset=[0 0 0]  TranslationCartesianOffsetUnits=m  TranslationStandardAxis=+Z  TranslationStandardOffset=0.1*1.5  TranslationStandardOffsetUnits=m  TranslationROffset=0  TranslationROffsetUnits=m  TranslationThetaOffset=0  TranslationThetaOffsetUnits=deg  TranslationZOffset=0  TranslationZOffsetUnits=m
  Simulink-PS Converter1 : nesl_utility/Simulink-PS Converter  PhysicalDomain=network_engine_domain  SubClassName=ps_input  LeftPortType=input  RightPortType=output  PseudoPeriodic=off  Frequencies=[]  NoiseDistribution=none  NoiseParameters=[]  Unit=rad  AffineConversion=off  FilteringAndDerivatives=filter  SimscapeFilterOrder=2  InputFilterTimeConstant=0.001  UdotUserProvided=0
  Sun ShaftA : Multibody_Parts_Lib/Basic/Rod  rod_rad=cvtPar.rad_hole*2  rod_len=0.1*1.5  rod_rho=7000  rod_color=cvtPar.clr.pg1.sun  rod_opc=1  popup_zori=Local +Z  popup_markings=None  mark_radius_range=[0.5 1.01]  mark_length_range=1.005  mark_angle_range=30  mark_color=[1 1 1]
  Sun ShaftB : Multibody_Parts_Lib/Basic/Rod  rod_rad=cvtPar.rad_hole*2  rod_len=0.1*1.5  rod_rho=7000  rod_color=cvtPar.clr.pg1.sun  rod_opc=1  popup_zori=Local +Z  popup_markings=None  mark_radius_range=[0.5 1.01]  mark_length_range=1.005  mark_angle_range=30  mark_color=[1 1 1]
  rpm 2 radps : Gain  Gain=2*pi/60
  T : PMIOPort  Side=Right
  W : PMIOPort  Port=2  Side=Right
  wires:
  w/1 -> rpm 2 radps/1
  Integrator/1 -> Simulink-PS Converter1/1
  rpm 2 radps/1 -> Integrator/1
  connections:
  W/RConn1 -- Rigid Transform/RConn1 -- Revolute/LConn1
  Revolute/RConn1 -- Sun ShaftA/RConn1 -- T/RConn1
  Revolute/RConn2 -- PS Terminator/LConn1
  Simulink-PS Converter1/RConn1 -- Revolute/LConn2
  Sun ShaftA/LConn1 -- Gear Assembly/LConn2 -- Sun ShaftB/RConn1
  Rigid Transform/LConn1 -- Gear Assembly/LConn3
  Motor/RConn1 -- Gear Assembly/LConn1

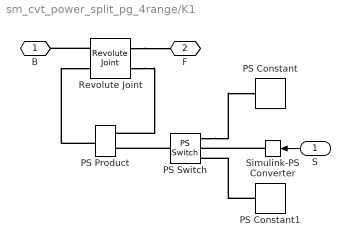
== system sm_cvt_power_split_pg_4range/K1 ==
  S : Inport
  PS Constant : fl_lib/Physical Signals/Sources/PS Constant  constant=-10000000 N*m*s/rad
  PS Constant1 : fl_lib/Physical Signals/Sources/PS Constant  constant=0 N*m*s/rad
  PS Product : fl_lib/Physical Signals/Functions/PS Product
  PS Switch : fl_lib/Physical Signals/Nonlinear Operators/PS Switch  Threshold=0.5  ZeroCross=true
      settings: InternalSimscapePortConfiguration="{\"Bottom\":[],\"Left\":[{\"id\":\"I1\",\"label\":\"\",\"type\":\"input\"},{\"id\":\"I2\",\"label\":\"\",\"type\":\"input\"},{\"id\":\"I3\",\"label\":\"\",\"type\":\"input\"}],\"Right\":[{\"id\":\"O\",\"label\":\"\",\"type\":\"output\"}],\"Top\":[]}"
  Revolute Joint : sm_lib/Joints/Revolute Joint  JointMode=Normal  CompositeWrenchDir=FollowerOnBase  CompositeWrenchFrame=BaseFrame  SenseConstraintForce=off  SenseConstraintTorque=off  SenseTotalForce=off  SenseTotalTorque=off  PositionTargetSpecify=off  PositionTargetPriority=High  PositionTargetValue=0  PositionTargetValueUnits=deg  VelocityTargetSpecify=off  VelocityTargetPriority=High  VelocityTargetValue=0  VelocityTargetValueUnits=deg/s  EquilibriumPosition=0  EquilibriumPositionUnits=deg  SpringStiffness=0  SpringStiffnessUnits=N*m/deg  DampingCoefficient=0  DampingCoefficientUnits=N*m/(deg/s)  LowerLimitSpecify=off  LowerLimitBound=-90  LowerLimitBoundUnits=deg  LowerLimitStiffness=1e4  LowerLimitStiffnessUnits=N*m/deg  LowerLimitDamping=10  LowerLimitDampingUnits=N*m/(deg/s)  LowerLimitTransitionRegionWidth=0.1  LowerLimitTransitionRegionWidthUnits=deg  UpperLimitSpecify=off  UpperLimitBound=90  UpperLimitBoundUnits=deg  UpperLimitStiffness=1e4  UpperLimitStiffnessUnits=N*m/deg  UpperLimitDamping=10  UpperLimitDampingUnits=N*m/(deg/s)  UpperLimitTransitionRegionWidth=0.1  UpperLimitTransitionRegionWidthUnits=deg  TorqueActuationMode=InputTorque  MotionActuationMode=ComputedMotion  SensePosition=off  SenseVelocity=on  SenseAcceleration=off  SenseTorqueForce=off  SenseLowerLimitTorqueForce=off  SenseUpperLimitTorqueForce=off
  Simulink-PS Converter : nesl_utility/Simulink-PS Converter  PhysicalDomain=network_engine_domain  SubClassName=ps_input  LeftPortType=input  RightPortType=output  PseudoPeriodic=off  Frequencies=[]  NoiseDistribution=none  NoiseParameters=[]  Unit=1  AffineConversion=off  FilteringAndDerivatives=provide  SimscapeFilterOrder=1  InputFilterTimeConstant=0.001  UdotUserProvided=0
  B : PMIOPort  Side=Left
  F : PMIOPort  Port=2  Side=Right
  wires:
  S/1 -> Simulink-PS Converter/1
  connections:
  Simulink-PS Converter/RConn1 -- PS Switch/LConn2
  PS Constant1/RConn1 -- PS Switch/LConn3
  PS Switch/LConn1 -- PS Constant/RConn1
  PS Switch/RConn1 -- PS Product/LConn2
  PS Product/RConn1 -- Revolute Joint/LConn2
  Revolute Joint/RConn2 -- PS Product/LConn1
  Revolute Joint/RConn1 -- F/RConn1
  Revolute Joint/LConn1 -- B/RConn1

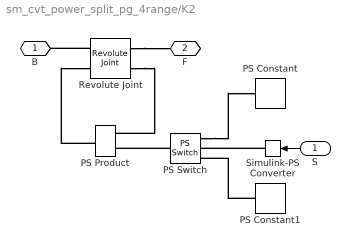
== system sm_cvt_power_split_pg_4range/K2 ==
  S : Inport
  PS Constant : fl_lib/Physical Signals/Sources/PS Constant  constant=-10000000 N*m*s/rad
  PS Constant1 : fl_lib/Physical Signals/Sources/PS Constant  constant=0 N*m*s/rad
  PS Product : fl_lib/Physical Signals/Functions/PS Product
  PS Switch : fl_lib/Physical Signals/Nonlinear Operators/PS Switch  Threshold=0.5  ZeroCross=true
      settings: InternalSimscapePortConfiguration="{\"Bottom\":[],\"Left\":[{\"id\":\"I1\",\"label\":\"\",\"type\":\"input\"},{\"id\":\"I2\",\"label\":\"\",\"type\":\"input\"},{\"id\":\"I3\",\"label\":\"\",\"type\":\"input\"}],\"Right\":[{\"id\":\"O\",\"label\":\"\",\"type\":\"output\"}],\"Top\":[]}"
  Revolute Joint : sm_lib/Joints/Revolute Joint  JointMode=Normal  CompositeWrenchDir=FollowerOnBase  CompositeWrenchFrame=BaseFrame  SenseConstraintForce=off  SenseConstraintTorque=off  SenseTotalForce=off  SenseTotalTorque=off  PositionTargetSpecify=off  PositionTargetPriority=High  PositionTargetValue=0  PositionTargetValueUnits=deg  VelocityTargetSpecify=off  VelocityTargetPriority=High  VelocityTargetValue=0  VelocityTargetValueUnits=deg/s  EquilibriumPosition=0  EquilibriumPositionUnits=deg  SpringStiffness=0  SpringStiffnessUnits=N*m/deg  DampingCoefficient=0  DampingCoefficientUnits=N*m/(deg/s)  LowerLimitSpecify=off  LowerLimitBound=-90  LowerLimitBoundUnits=deg  LowerLimitStiffness=1e4  LowerLimitStiffnessUnits=N*m/deg  LowerLimitDamping=10  LowerLimitDampingUnits=N*m/(deg/s)  LowerLimitTransitionRegionWidth=0.1  LowerLimitTransitionRegionWidthUnits=deg  UpperLimitSpecify=off  UpperLimitBound=90  UpperLimitBoundUnits=deg  UpperLimitStiffness=1e4  UpperLimitStiffnessUnits=N*m/deg  UpperLimitDamping=10  UpperLimitDampingUnits=N*m/(deg/s)  UpperLimitTransitionRegionWidth=0.1  UpperLimitTransitionRegionWidthUnits=deg  TorqueActuationMode=InputTorque  MotionActuationMode=ComputedMotion  SensePosition=off  SenseVelocity=on  SenseAcceleration=off  SenseTorqueForce=off  SenseLowerLimitTorqueForce=off  SenseUpperLimitTorqueForce=off
  Simulink-PS Converter : nesl_utility/Simulink-PS Converter  PhysicalDomain=network_engine_domain  SubClassName=ps_input  LeftPortType=input  RightPortType=output  PseudoPeriodic=off  Frequencies=[]  NoiseDistribution=none  NoiseParameters=[]  Unit=1  AffineConversion=off  FilteringAndDerivatives=provide  SimscapeFilterOrder=1  InputFilterTimeConstant=0.001  UdotUserProvided=0
  B : PMIOPort  Side=Left
  F : PMIOPort  Port=2  Side=Right
  wires:
  S/1 -> Simulink-PS Converter/1
  connections:
  Revolute Joint/LConn1 -- B/RConn1
  Revolute Joint/RConn1 -- F/RConn1
  Revolute Joint/RConn2 -- PS Product/LConn1
  PS Product/RConn1 -- Revolute Joint/LConn2
  PS Switch/RConn1 -- PS Product/LConn2
  PS Switch/LConn1 -- PS Constant/RConn1
  PS Constant1/RConn1 -- PS Switch/LConn3
  Simulink-PS Converter/RConn1 -- PS Switch/LConn2

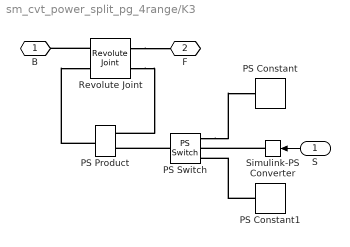
== system sm_cvt_power_split_pg_4range/K3 ==
  S : Inport
  PS Constant : fl_lib/Physical Signals/Sources/PS Constant  constant=-10000000 N*m*s/rad
  PS Constant1 : fl_lib/Physical Signals/Sources/PS Constant  constant=0 N*m*s/rad
  PS Product : fl_lib/Physical Signals/Functions/PS Product
  PS Switch : fl_lib/Physical Signals/Nonlinear Operators/PS Switch  Threshold=0.5  ZeroCross=true
      settings: InternalSimscapePortConfiguration="{\"Bottom\":[],\"Left\":[{\"id\":\"I1\",\"label\":\"\",\"type\":\"input\"},{\"id\":\"I2\",\"label\":\"\",\"type\":\"input\"},{\"id\":\"I3\",\"label\":\"\",\"type\":\"input\"}],\"Right\":[{\"id\":\"O\",\"label\":\"\",\"type\":\"output\"}],\"Top\":[]}"
  Revolute Joint : sm_lib/Joints/Revolute Joint  JointMode=Normal  CompositeWrenchDir=FollowerOnBase  CompositeWrenchFrame=BaseFrame  SenseConstraintForce=off  SenseConstraintTorque=off  SenseTotalForce=off  SenseTotalTorque=off  PositionTargetSpecify=off  PositionTargetPriority=High  PositionTargetValue=0  PositionTargetValueUnits=deg  VelocityTargetSpecify=off  VelocityTargetPriority=High  VelocityTargetValue=0  VelocityTargetValueUnits=deg/s  EquilibriumPosition=0  EquilibriumPositionUnits=deg  SpringStiffness=0  SpringStiffnessUnits=N*m/deg  DampingCoefficient=0  DampingCoefficientUnits=N*m/(deg/s)  LowerLimitSpecify=off  LowerLimitBound=-90  LowerLimitBoundUnits=deg  LowerLimitStiffness=1e4  LowerLimitStiffnessUnits=N*m/deg  LowerLimitDamping=10  LowerLimitDampingUnits=N*m/(deg/s)  LowerLimitTransitionRegionWidth=0.1  LowerLimitTransitionRegionWidthUnits=deg  UpperLimitSpecify=off  UpperLimitBound=90  UpperLimitBoundUnits=deg  UpperLimitStiffness=1e4  UpperLimitStiffnessUnits=N*m/deg  UpperLimitDamping=10  UpperLimitDampingUnits=N*m/(deg/s)  UpperLimitTransitionRegionWidth=0.1  UpperLimitTransitionRegionWidthUnits=deg  TorqueActuationMode=InputTorque  MotionActuationMode=ComputedMotion  SensePosition=off  SenseVelocity=on  SenseAcceleration=off  SenseTorqueForce=off  SenseLowerLimitTorqueForce=off  SenseUpperLimitTorqueForce=off
  Simulink-PS Converter : nesl_utility/Simulink-PS Converter  PhysicalDomain=network_engine_domain  SubClassName=ps_input  LeftPortType=input  RightPortType=output  PseudoPeriodic=off  Frequencies=[]  NoiseDistribution=none  NoiseParameters=[]  Unit=1  AffineConversion=off  FilteringAndDerivatives=provide  SimscapeFilterOrder=1  InputFilterTimeConstant=0.001  UdotUserProvided=0
  B : PMIOPort  Side=Left
  F : PMIOPort  Port=2  Side=Right
  wires:
  S/1 -> Simulink-PS Converter/1
  connections:
  Simulink-PS Converter/RConn1 -- PS Switch/LConn2
  PS Constant1/RConn1 -- PS Switch/LConn3
  PS Switch/LConn1 -- PS Constant/RConn1
  PS Switch/RConn1 -- PS Product/LConn2
  PS Product/RConn1 -- Revolute Joint/LConn2
  Revolute Joint/RConn2 -- PS Product/LConn1
  Revolute Joint/RConn1 -- F/RConn1
  Revolute Joint/LConn1 -- B/RConn1

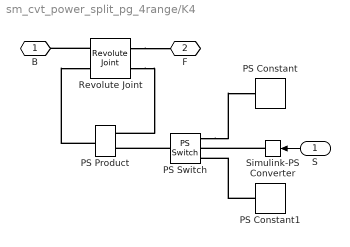
== system sm_cvt_power_split_pg_4range/K4 ==
  S : Inport
  PS Constant : fl_lib/Physical Signals/Sources/PS Constant  constant=-10000000 N*m*s/rad
  PS Constant1 : fl_lib/Physical Signals/Sources/PS Constant  constant=0 N*m*s/rad
  PS Product : fl_lib/Physical Signals/Functions/PS Product
  PS Switch : fl_lib/Physical Signals/Nonlinear Operators/PS Switch  Threshold=0.5  ZeroCross=true
      settings: InternalSimscapePortConfiguration="{\"Bottom\":[],\"Left\":[{\"id\":\"I1\",\"label\":\"\",\"type\":\"input\"},{\"id\":\"I2\",\"label\":\"\",\"type\":\"input\"},{\"id\":\"I3\",\"label\":\"\",\"type\":\"input\"}],\"Right\":[{\"id\":\"O\",\"label\":\"\",\"type\":\"output\"}],\"Top\":[]}"
  Revolute Joint : sm_lib/Joints/Revolute Joint  JointMode=Normal  CompositeWrenchDir=FollowerOnBase  CompositeWrenchFrame=BaseFrame  SenseConstraintForce=off  SenseConstraintTorque=off  SenseTotalForce=off  SenseTotalTorque=off  PositionTargetSpecify=off  PositionTargetPriority=High  PositionTargetValue=0  PositionTargetValueUnits=deg  VelocityTargetSpecify=off  VelocityTargetPriority=High  VelocityTargetValue=0  VelocityTargetValueUnits=deg/s  EquilibriumPosition=0  EquilibriumPositionUnits=deg  SpringStiffness=0  SpringStiffnessUnits=N*m/deg  DampingCoefficient=0  DampingCoefficientUnits=N*m/(deg/s)  LowerLimitSpecify=off  LowerLimitBound=-90  LowerLimitBoundUnits=deg  LowerLimitStiffness=1e4  LowerLimitStiffnessUnits=N*m/deg  LowerLimitDamping=10  LowerLimitDampingUnits=N*m/(deg/s)  LowerLimitTransitionRegionWidth=0.1  LowerLimitTransitionRegionWidthUnits=deg  UpperLimitSpecify=off  UpperLimitBound=90  UpperLimitBoundUnits=deg  UpperLimitStiffness=1e4  UpperLimitStiffnessUnits=N*m/deg  UpperLimitDamping=10  UpperLimitDampingUnits=N*m/(deg/s)  UpperLimitTransitionRegionWidth=0.1  UpperLimitTransitionRegionWidthUnits=deg  TorqueActuationMode=InputTorque  MotionActuationMode=ComputedMotion  SensePosition=off  SenseVelocity=on  SenseAcceleration=off  SenseTorqueForce=off  SenseLowerLimitTorqueForce=off  SenseUpperLimitTorqueForce=off
  Simulink-PS Converter : nesl_utility/Simulink-PS Converter  PhysicalDomain=network_engine_domain  SubClassName=ps_input  LeftPortType=input  RightPortType=output  PseudoPeriodic=off  Frequencies=[]  NoiseDistribution=none  NoiseParameters=[]  Unit=1  AffineConversion=off  FilteringAndDerivatives=provide  SimscapeFilterOrder=1  InputFilterTimeConstant=0.001  UdotUserProvided=0
  B : PMIOPort  Side=Left
  F : PMIOPort  Port=2  Side=Right
  wires:
  S/1 -> Simulink-PS Converter/1
  connections:
  Revolute Joint/LConn1 -- B/RConn1
  Revolute Joint/RConn1 -- F/RConn1
  Revolute Joint/RConn2 -- PS Product/LConn1
  PS Product/RConn1 -- Revolute Joint/LConn2
  PS Switch/RConn1 -- PS Product/LConn2
  PS Switch/LConn1 -- PS Constant/RConn1
  PS Constant1/RConn1 -- PS Switch/LConn3
  Simulink-PS Converter/RConn1 -- PS Switch/LConn2

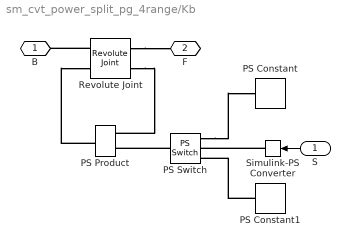
== system sm_cvt_power_split_pg_4range/Kb ==
  S : Inport
  PS Constant : fl_lib/Physical Signals/Sources/PS Constant  constant=-10000000 N*m*s/rad
  PS Constant1 : fl_lib/Physical Signals/Sources/PS Constant  constant=0 N*m*s/rad
  PS Product : fl_lib/Physical Signals/Functions/PS Product
  PS Switch : fl_lib/Physical Signals/Nonlinear Operators/PS Switch  Threshold=0.5  ZeroCross=true
      settings: InternalSimscapePortConfiguration="{\"Bottom\":[],\"Left\":[{\"id\":\"I1\",\"label\":\"\",\"type\":\"input\"},{\"id\":\"I2\",\"label\":\"\",\"type\":\"input\"},{\"id\":\"I3\",\"label\":\"\",\"type\":\"input\"}],\"Right\":[{\"id\":\"O\",\"label\":\"\",\"type\":\"output\"}],\"Top\":[]}"
  Revolute Joint : sm_lib/Joints/Revolute Joint  JointMode=Normal  CompositeWrenchDir=FollowerOnBase  CompositeWrenchFrame=BaseFrame  SenseConstraintForce=off  SenseConstraintTorque=off  SenseTotalForce=off  SenseTotalTorque=off  PositionTargetSpecify=off  PositionTargetPriority=High  PositionTargetValue=0  PositionTargetValueUnits=deg  VelocityTargetSpecify=off  VelocityTargetPriority=High  VelocityTargetValue=0  VelocityTargetValueUnits=deg/s  EquilibriumPosition=0  EquilibriumPositionUnits=deg  SpringStiffness=0  SpringStiffnessUnits=N*m/deg  DampingCoefficient=0  DampingCoefficientUnits=N*m/(deg/s)  LowerLimitSpecify=off  LowerLimitBound=-90  LowerLimitBoundUnits=deg  LowerLimitStiffness=1e4  LowerLimitStiffnessUnits=N*m/deg  LowerLimitDamping=10  LowerLimitDampingUnits=N*m/(deg/s)  LowerLimitTransitionRegionWidth=0.1  LowerLimitTransitionRegionWidthUnits=deg  UpperLimitSpecify=off  UpperLimitBound=90  UpperLimitBoundUnits=deg  UpperLimitStiffness=1e4  UpperLimitStiffnessUnits=N*m/deg  UpperLimitDamping=10  UpperLimitDampingUnits=N*m/(deg/s)  UpperLimitTransitionRegionWidth=0.1  UpperLimitTransitionRegionWidthUnits=deg  TorqueActuationMode=InputTorque  MotionActuationMode=ComputedMotion  SensePosition=off  SenseVelocity=on  SenseAcceleration=off  SenseTorqueForce=off  SenseLowerLimitTorqueForce=off  SenseUpperLimitTorqueForce=off
  Simulink-PS Converter : nesl_utility/Simulink-PS Converter  PhysicalDomain=network_engine_domain  SubClassName=ps_input  LeftPortType=input  RightPortType=output  PseudoPeriodic=off  Frequencies=[]  NoiseDistribution=none  NoiseParameters=[]  Unit=1  AffineConversion=off  FilteringAndDerivatives=provide  SimscapeFilterOrder=1  InputFilterTimeConstant=0.001  UdotUserProvided=0
  B : PMIOPort  Side=Left
  F : PMIOPort  Port=2  Side=Right
  wires:
  S/1 -> Simulink-PS Converter/1
  connections:
  Revolute Joint/LConn1 -- B/RConn1
  Revolute Joint/RConn1 -- F/RConn1
  Revolute Joint/RConn2 -- PS Product/LConn1
  PS Product/RConn1 -- Revolute Joint/LConn2
  PS Switch/RConn1 -- PS Product/LConn2
  PS Switch/LConn1 -- PS Constant/RConn1
  PS Constant1/RConn1 -- PS Switch/LConn3
  Simulink-PS Converter/RConn1 -- PS Switch/LConn2

== system sm_cvt_power_split_pg_4range/Output Shaft ==
  Rigid Transform : sm_lib/Frames and Transforms/Rigid Transform  RotationMethod=None  FollAlignAxisA=+X  BaseAlignAxisA=+Y  FollAlignAxisB=+Y  BaseAlignAxisB=+Z  RotationStandardAxis=+Z  RotationAngle=0.0  RotationAngleUnits=deg  RotationArbitraryAxis=[0 0 1]  RotationSequenceAxes=FollowerAxes  RotationSequence=XYX  RotationSequenceAngles=[0 0 0]  RotationSequenceAnglesUnits=deg  RotationMatrix=[1 0 0; 0 1 0; 0 0 1]  Quaternion=[1 0 0 0]  TranslationMethod=StandardAxis  TranslationCartesianOffset=[0 0 0]  TranslationCartesianOffsetUnits=m  TranslationStandardAxis=+Z  TranslationStandardOffset=-cvtPar.plaGear_axial_offset+cvtPar.gear_thickness  TranslationStandardOffsetUnits=m  TranslationROffset=0  TranslationROffsetUnits=m  TranslationThetaOffset=0  TranslationThetaOffsetUnits=deg  TranslationZOffset=0  TranslationZOffsetUnits=m
  Rod Sun : Multibody_Parts_Lib/Basic/Rod  rod_rad=cvtPar.rad_hole*2  rod_len=cvtPar.gear_thickness*2  rod_rho=7000  rod_color=cvtPar.clr.pg4.carr  rod_opc=1  popup_zori=Local +Z  popup_markings=None  mark_radius_range=[0.5 1.01]  mark_length_range=1.005  mark_angle_range=30  mark_color=[1 1 1]
  F : PMIOPort  Side=Right
  connections:
  Rigid Transform/LConn1 -- F/RConn1
  Rod Sun/LConn1 -- Rigid Transform/RConn1

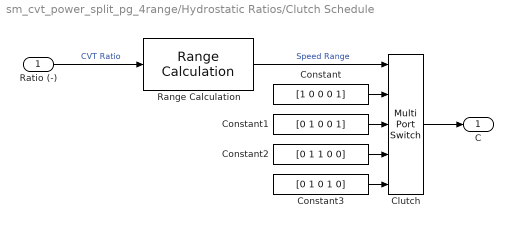
== system sm_cvt_power_split_pg_4range/Hydrostatic Ratios/Clutch Schedule ==
  Ratio (-) : Inport
  Clutch : MultiPortSwitch  Inputs=4  SaturateOnIntegerOverflow=off  InputSameDT=off
  Constant : Constant  Value=[1 0 0 0 1]
  Constant1 : Constant  Value=[0 1 0 0 1]
  Constant2 : Constant  Value=[0 1 1 0 0]
  Constant3 : Constant  Value=[0 1 0 1 0]
  Range Calculation : sm_wheel_loader_lib/Controller/CVT Ratio Ctrl/Range Calculation  XY_I=HMPST.Ctrl.Swash.XY_I
  C : Outport
  wires:
  Ratio (-)/1 -> Range Calculation/1  "CVT Ratio"
  Constant1/1 -> Clutch/3
  Constant2/1 -> Clutch/4
  Clutch/1 -> C/1
  Constant3/1 -> Clutch/5
  Constant/1 -> Clutch/2
  Range Calculation/1 -> Clutch/1  "Speed Range"
